simulink library "WECSim_Lib_Body_Elements"  (R2020b)
settings: Solver=VariableStepAuto  StartTime=0.0  StopTime=10.0  RelTol=1e-3
undefined symbols (not defined in the file or in its folder): body, simu, waves, X, Y, Z
libraries: nesl_utility x22, sm_lib x16, $bdroot x9, vrlib x3
(part 2 of 5)

== system WECSim_Lib_Body_Elements/Flex Body/Variable Hydrodynamics Control ==
  note: Developer note: When creating a new bus selector, it will only show the variables within hydroForce if they already exist in the workspace, which is inconventient. Copy this bus selector to more easily add calls to variables from hydroForce. This bus selector should already contains all variables in hydroForce which can then be selected, and extras deleted.
      |
      | Alternatively, open the bus selector block and use programmatic commands to set the output variables, e.g.
      | >> set_param(gcb, 'OutputSignals', 'storage.mass, volume');
  Bus Selector : BusSelector  Commented=on  OutputSignals=linearHydroRestCoef,storage,quadDrag,linearDamping,fExt,fExt.re,fExt.im,fExt.md,fAddedMass,fDamping,irkb,storage.mass,storage.inertia,storage.inertiaProducts,storage.fAddedMass,userDefinedFe,totDOF,fExt.dofGrd,fExt.dirGrd,fExt.wGrd,fExt.fEHRE,fExt.fEHIM,fExt.fEHMD
  Constant : Constant  Value=body.hydroForce  VectorParams1D=off  OutDataTypeStr=Bus: bus_body1_hydroForce
  From : From  Commented=on  GotoTag=body1_hydroForce
  Variable Hydrodynamics Subsystem : Subsystem  Variant=on  VariantControl=sv_b1_variableHydro  mask{body=body}
  tag scope: body1_hydroForce=global
  wires:
  Constant/1 -> Variable Hydrodynamics Subsystem/1(all_hydroForce)
  Variable Hydrodynamics Subsystem/1(selected_hydroForce) -> [body1_hydroForce]
  From/1 -> Bus Selector/1

== system WECSim_Lib_Body_Elements/Flex Body/Wave Diffraction and Excitation Force Calculation ==
  note: Do not link the `Wave Diffraction and Excitation Force Calculation`
      | to the rigid body block, this will break the Flex Body block.
  Time : Inport
  Displacement : Inport  Port=2
  WaveElv : Inport  Port=3
  Selector : Selector  InputPortWidth=body.dof  IndexOptions=Index vector (dialog)  Indices=[1:6]  OutputSizes=1
  Selector1 : Selector  InputPortWidth=body.dof  IndexOptions=Index vector (dialog)  Indices=[7:body.dofEnd]  OutputSizes=1
  Wave Diffraction and Excitation Force Calculation : Subsystem  mask{waveGroup=0}
      mask prompts: waveGroup "Waves Object"
      mask init:
      | cb = gcb;
      | nWaves = size(waveGroup,2);
      | for iWG = 2:nWaves
      |     try 
      |         find_system([cb,'/Linear Wave Excitation Force Variant Subsystem',num2str(iWG)],'Type','Block');
      |     catch
      |         add_block([cb,'/Linear Wave Excitation Force Variant Subsystem'],[cb,'/Wave Diffraction and Excitation Force Calculation/Linear Wave Excitation Force Variant Subsystem',num2str(iWG)],'MakeNameUnique','off',...
      |                    'Position',[400,200*iWG,580,40+200*iWG],'BackgroundColor','white');
      |         set_param([cb,'/Linear Wave Excitation Force Variant Subsystem',num2str(iWG)],...
      |                'Nwave',sprintf('waves(%d)',iWG) );
      | 
      |         add_line(cb,...
      |            ['FexcInputs/1'],...
      |             ['Linear Wave Excitation Force Variant Subsystem',num2str(iWG),'/1'],...
      |             'autorouting','on');
      |            add_line(cb,...
      |            ['FexcInputs/2'],...
      |             ['Linear Wave Excitation Force Variant Subsystem',num2str(iWG),'/2'],...
      |             'autorouting','on');
      |         signlist = get_param([cb,'/Add'],'Inputs');   
      |         set_param([cb,'/Add'],'Inputs',[signlist,'+']);
      |         add_line(cb,...
      |         ['Linear Wave Excitation Force Variant Subsystem',num2str(iWG),'/1'],...
      |         sprintf('Add/%d',length(signlist)+1),...
      |         'autorouting','on');
      |     end
      | end
  F_Excitation_Rigid : Outport  PortDimensions=6
  F_Excitation_Flex : Outport  Port=2  PortDimensions=body.gbmDOF
  wires:
  Displacement/1 -> Wave Diffraction and Excitation Force Calculation/2(Displacement)
  WaveElv/1 -> Wave Diffraction and Excitation Force Calculation/3(WaveElv)
  Time/1 -> Wave Diffraction and Excitation Force Calculation/1(Time)
  Selector1/1 -> F_Excitation_Flex/1
  Selector/1 -> F_Excitation_Rigid/1
  Wave Diffraction and Excitation Force Calculation/1(F_Excitation) -> Selector/1, Selector1/1

== system WECSim_Lib_Body_Elements/Flex Body/Wave Radiation Forces Calculation ==
  Velocity : Inport
  Acceleration : Inport  Port=2
  Selector : Selector  InputPortWidth=body.dof  IndexOptions=Index vector (dialog)  Indices=[1:6]  OutputSizes=1
  Selector1 : Selector  InputPortWidth=body.dof  IndexOptions=Index vector (dialog)  Indices=[7:body.dofEnd]  OutputSizes=1
  Selector2 : Selector  InputPortWidth=body.dof  IndexOptions=Index vector (dialog)  Indices=[1:6]  OutputSizes=1
  Selector3 : Selector  InputPortWidth=body.dof  IndexOptions=Index vector (dialog)  Indices=[7:body.dofEnd]  OutputSizes=1
  Wave Radiation Forces Calculation : Subsystem  AncestorBlock=WECSim_Lib_Body_Elements/Rigid Body/Hydrodynamic Body/Wave Radiation Forces Calculation  mask{body=body}
      mask prompts: body "Body class:"
  F_RadiationDamping_Rigid : Outport  PortDimensions=6
  F_RadiationDamping_Flex : Outport  Port=2  PortDimensions=body.gbmDOF
  F_AddedMass_Rigid : Outport  Port=3  PortDimensions=6
  F_AddedMass_Flex : Outport  Port=4  PortDimensions=body.gbmDOF
  wires:
  Velocity/1 -> Wave Radiation Forces Calculation/1(Velocity)
  Acceleration/1 -> Wave Radiation Forces Calculation/2(Acceleration)
  Wave Radiation Forces Calculation/1(F_RadiationDamping) -> Selector1/1, Selector/1  "F_RadiationDamping"
  Selector1/1 -> F_RadiationDamping_Flex/1
  Selector/1 -> F_RadiationDamping_Rigid/1
  Selector3/1 -> F_AddedMass_Flex/1
  Selector2/1 -> F_AddedMass_Rigid/1
  Wave Radiation Forces Calculation/2(F_AddedMass) -> Selector2/1, Selector3/1  "F_AddedMass"

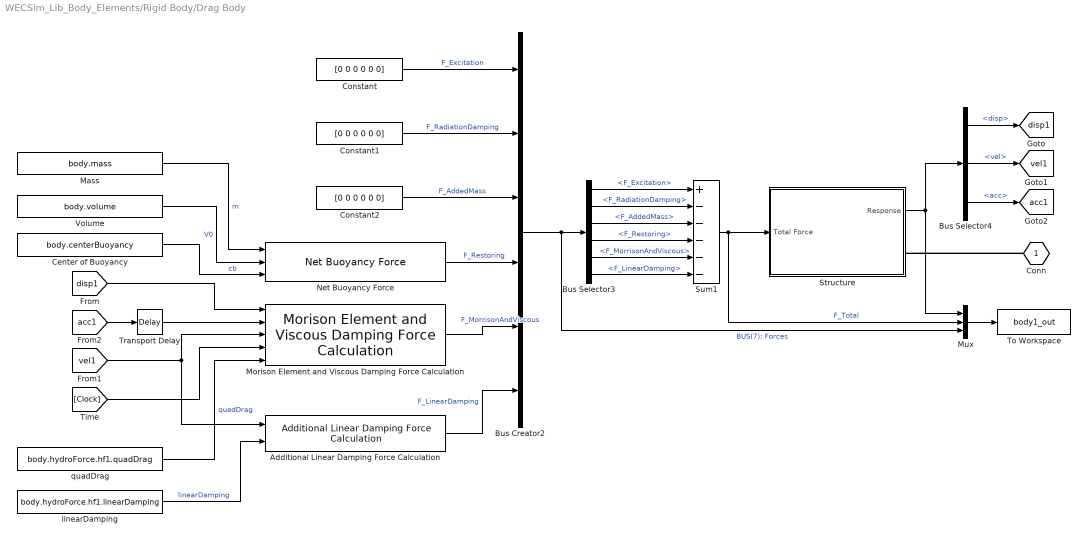
== system WECSim_Lib_Body_Elements/Rigid Body/Drag Body ==
  Additional Linear Damping Force Calculation : $bdroot/Rigid Body/Hydrodynamic Body/Additional Linear Damping Force Calculation  SystemSampleTime=-1  VariantActivationTime=update diagram  EmptyChoice=off  PassThrough=off  PassThroughVariantControl=(default)  EmptyChoiceVariantControl=(default)  Latency=0  AutoFrameSizeCalculation=off
  Bus Creator2 : BusCreator  Inputs=6
  Bus Selector3 : BusSelector  OutputSignals=F_Excitation,F_RadiationDamping,F_AddedMass,F_Restoring,F_MorrisonAndViscous,F_LinearDamping
  Bus Selector4 : BusSelector  OutputSignals=disp,vel,acc
  Center of Buoyancy : Constant  Value=body.centerBuoyancy
  Constant : Constant  Value=[0 0 0 0 0 0]
  Constant1 : Constant  Value=[0 0 0 0 0 0]
  Constant2 : Constant  Value=[0 0 0 0 0 0]
  Mass : Constant  Value=body.mass
  Morison Element and Viscous Damping Force Calculation : $bdroot/Rigid Body/Hydrodynamic Body/Morison Element and Viscous Damping Force Calculation  SystemSampleTime=-1  VariantActivationTime=update diagram  EmptyChoice=off  PassThrough=off  PassThroughVariantControl=(default)  EmptyChoiceVariantControl=(default)  Latency=0  AutoFrameSizeCalculation=off
  Mux : Mux  Inputs=3
  Net Buoyancy Force : $bdroot/Rigid Body/Hydrodynamic Body/Hydrostatic Restoring Force Calculation/Linear and Nonlinear Restoring Force Variant Subsystem/Linear Hydrostatic Restoring Force/Net Buoyancy Force  SystemSampleTime=-1  VariantActivationTime=update diagram  EmptyChoice=off  PassThrough=off  PassThroughVariantControl=(default)  EmptyChoiceVariantControl=(default)  Latency=0  AutoFrameSizeCalculation=off
  Structure : Subsystem
  Sum1 : Sum  Inputs=+-----
  To Workspace : ToWorkspace  VariableName=body1_out  SaveFormat=Structure With Time  SampleTime=simu.dtOut
  Transport Delay : TransportDelay  DelayTime=10e-8
  Volume : Constant  Value=body.volume
  linearDamping : Constant  Value=body.hydroForce.hf1.linearDamping
  quadDrag : Constant  Value=body.hydroForce.hf1.quadDrag
  Conn : PMIOPort  Side=Right
  tag scope: acc1=global, disp1=global, vel1=global
  wires:
  [acc1] -> Transport Delay/1
  Bus Selector3/1 -> Sum1/1  "<F_Excitation>"
  Bus Selector3/5 -> Sum1/5  "<F_MorrisonAndViscous>"
  Constant1/1 -> Bus Creator2/2  "F_RadiationDamping"
  Mux/1 -> To Workspace/1
  Net Buoyancy Force/1 -> Bus Creator2/4  "F_Restoring"
  Additional Linear Damping Force Calculation/1 -> Bus Creator2/6  "F_LinearDamping"
  Morison Element and Viscous Damping Force Calculation/1 -> Bus Creator2/5  "F_MorrisonAndViscous"
  Constant/1 -> Bus Creator2/1  "F_Excitation"
  Bus Selector3/4 -> Sum1/4  "<F_Restoring>"
  Bus Selector3/3 -> Sum1/3  "<F_AddedMass>"
  Bus Creator2/1 -> Mux/3, Bus Selector3/1  "BUS(7): Forces"
  Sum1/1 -> Mux/2, Structure/1(Total Force)  "F_Total"
  Constant2/1 -> Bus Creator2/3  "F_AddedMass"
  Bus Selector3/2 -> Sum1/2  "<F_RadiationDamping>"
  Bus Selector3/6 -> Sum1/6  "<F_LinearDamping>"
  Bus Selector4/1 -> [disp1]  "<disp>"
  Bus Selector4/2 -> [vel1]  "<vel>"
  Structure/1(Response) -> Mux/1, Bus Selector4/1
  Bus Selector4/3 -> [acc1]  "<acc>"
  Transport Delay/1 -> Morison Element and Viscous Damping Force Calculation/2
  [vel1] -> Morison Element and Viscous Damping Force Calculation/3, Additional Linear Damping Force Calculation/1
  [Clock] -> Morison Element and Viscous Damping Force Calculation/4
  [disp1] -> Morison Element and Viscous Damping Force Calculation/1
  Center of Buoyancy/1 -> Net Buoyancy Force/3  "cb"
  Volume/1 -> Net Buoyancy Force/2  "V0"
  Mass/1 -> Net Buoyancy Force/1  "m"
  quadDrag/1 -> Morison Element and Viscous Damping Force Calculation/5  "quadDrag"
  linearDamping/1 -> Additional Linear Damping Force Calculation/2  "linearDamping"
  connections:
  Conn/RConn1 -- Structure/RConn1

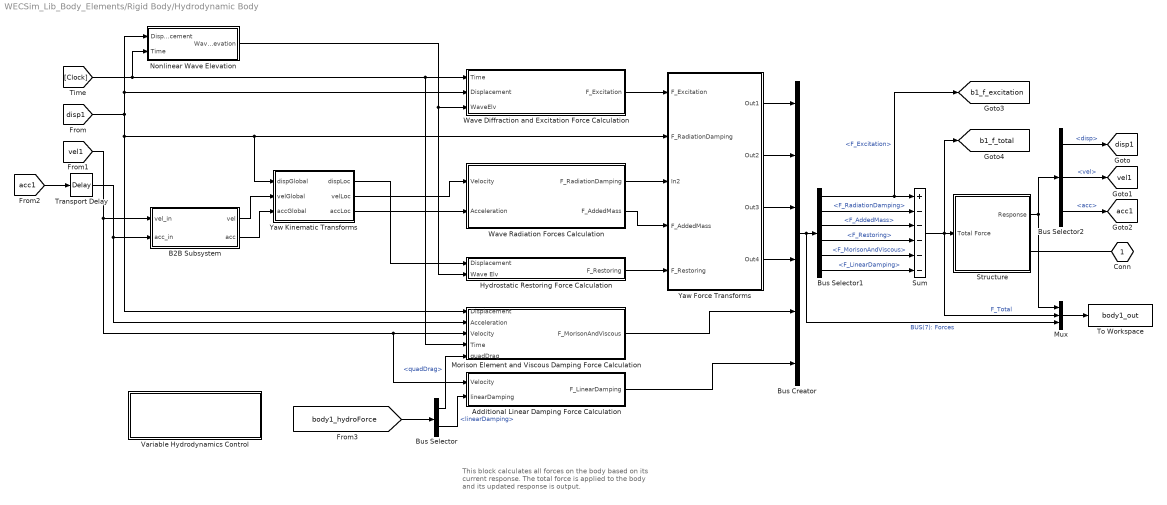
== system WECSim_Lib_Body_Elements/Rigid Body/Hydrodynamic Body ==
  note: This block calculates all forces on the body based on its current response. The total force is applied to the body and its updated response is output.
  Additional Linear Damping Force Calculation : Subsystem
  B2B Subsystem : Subsystem  Variant=on
  Bus Creator : BusCreator  Inputs=6
  Bus Selector : BusSelector  OutputSignals=quadDrag,linearDamping
  Bus Selector1 : BusSelector  OutputSignals=F_Excitation,F_RadiationDamping,F_AddedMass,F_Restoring,F_MorisonAndViscous,F_LinearDamping
  Bus Selector2 : BusSelector  OutputSignals=disp,vel,acc
  Hydrostatic Restoring Force Calculation : Subsystem
  Morison Element and Viscous Damping Force Calculation : Subsystem
  Mux : Mux  Inputs=3
  Nonlinear Wave Elevation : Subsystem  TreatAsAtomicUnit=on  SystemSampleTime=simu.nonlinearDt
  Structure : Subsystem
  Sum : Sum  Inputs=+-----
  To Workspace : ToWorkspace  VariableName=body1_out  SaveFormat=Structure With Time  SampleTime=simu.dtOut
  Transport Delay : TransportDelay  DelayTime=10e-8
  Variable Hydrodynamics Control : Subsystem  mask{body=body}
      mask prompts: body "Body Name:"
  Wave Diffraction and Excitation Force Calculation : Subsystem  mask{waveGroup=waves}
      mask prompts: waveGroup "Waves Object"
      mask init:
      | cb = gcb;
      | nWaves = size(waveGroup,2);
      | for iWG = 2:nWaves
      |     try 
      |         find_system([cb,'/Linear Wave Excitation Force Variant Subsystem',num2str(iWG)],'Type','Block');
      |     catch
      |         % Duplicate the linear excitation force block for multiple waves
      |         add_block([cb,'/Linear Wave Excitation Force Variant Subsystem'],[cb,'/Linear Wave Excitation Force Variant Subsystem',num2str(iWG)],'MakeNameUnique','off',...
      |                    'Position',[400,200*iWG,580,40+200*iWG],'BackgroundColor','white');
      |         set_param([cb,'/Linear Wave Excitation Force Variant Subsystem',num2str(iWG)],...
      |                'Nwave',sprintf('waves(%d)',iWG) );
      | 
      |         % Connect lines to the new block
      |         add_line(cb,...
      |            ['FexcInputs/1'],...
      |            ['Linear Wave Excitation Force Variant Subsystem',num2str(iWG),'/1'],...
      |            'autorouting','on');
      |         add_line(cb,...
      |            ['FexcInputs/2'],...
      |            ['Linear Wave Excitation Force Variant Subsystem',num2str(iWG),'/2'],...
      |            'autorouting','on');
      |         add_line(cb,...
      |            ['FexcInputs/4'],...
      |            ['Linear Wave Excitation Force Variant Subsystem',num2str(iWG),'/3'],...
      |            'autorouting','on');
      |         signlist = get_param([cb,'/Add'],'Inputs');   
      |         set_param([cb,'/Add'],'Inputs',[signlist,'+']);
      |         add_line(cb,...
      |         ['Linear Wave Excitation Force Variant Subsystem',num2str(iWG),'/1'],...
      |         sprintf('Add/%d',length(signlist)+1),...
      |         'autorouting','on');
      |     end
      | end
  Wave Radiation Forces Calculation : Subsystem
  Yaw Force Transforms : Subsystem
  Yaw Kinematic Transforms : Subsystem  Variant=on
  Conn : PMIOPort  Side=Right
  tag scope: acc1=global, b1_f_excitation=global, b1_f_total=global, disp1=global, vel1=global
  wires:
  Bus Selector1/6 -> Sum/6  "<F_LinearDamping>"
  Bus Selector1/5 -> Sum/5  "<F_MorisonAndViscous>"
  Bus Selector1/4 -> Sum/4  "<F_Restoring>"
  Bus Selector1/3 -> Sum/3  "<F_AddedMass>"
  Bus Selector1/2 -> Sum/2  "<F_RadiationDamping>"
  Bus Selector1/1 -> [b1_f_excitation], Sum/1  "<F_Excitation>"
  Hydrostatic Restoring Force Calculation/1(F_Restoring) -> Yaw Force Transforms/5(F_Restoring)
  [disp1] -> Nonlinear Wave Elevation/1(Displacement), Wave Diffraction and Excitation Force Calculation/2(Displacement), Yaw Kinematic Transforms/1(dispGlobal), Yaw Force Transforms/2(F_RadiationDamping), Morison Element and Viscous Damping Force Calculation/1(Displacement)
  Wave Diffraction and Excitation Force Calculation/1(F_Excitation) -> Yaw Force Transforms/1(F_Excitation)
  Wave Radiation Forces Calculation/2(F_AddedMass) -> Yaw Force Transforms/4(F_AddedMass)
  Morison Element and Viscous Damping Force Calculation/1(F_MorisonAndViscous) -> Bus Creator/5
  Structure/1(Response) -> Mux/1, Bus Selector2/1
  Bus Creator/1 -> Mux/3, Bus Selector1/1  "BUS(7): Forces"
  B2B Subsystem/2(acc) -> Yaw Kinematic Transforms/3(accGlobal)
  Bus Selector2/2 -> [vel1]  "<vel>"
  Sum/1 -> [b1_f_total], Mux/2, Structure/1(Total Force)  "F_Total"
  Bus Selector2/1 -> [disp1]  "<disp>"
  [acc1] -> Transport Delay/1
  Yaw Kinematic Transforms/3(accLoc) -> Wave Radiation Forces Calculation/2(Acceleration)
  [Clock] -> Nonlinear Wave Elevation/2(Time), Wave Diffraction and Excitation Force Calculation/1(Time), Morison Element and Viscous Damping Force Calculation/4(Time)
  Additional Linear Damping Force Calculation/1(F_LinearDamping) -> Bus Creator/6
  Transport Delay/1 -> B2B Subsystem/2(acc_in), Morison Element and Viscous Damping Force Calculation/2(Acceleration)
  Bus Selector2/3 -> [acc1]  "<acc>"
  B2B Subsystem/1(vel) -> Yaw Kinematic Transforms/2(velGlobal)
  Yaw Kinematic Transforms/1(dispLoc) -> Hydrostatic Restoring Force Calculation/1(Displacement)
  Yaw Kinematic Transforms/2(velLoc) -> Wave Radiation Forces Calculation/1(Velocity)
  Nonlinear Wave Elevation/1(Wave Elevation) -> Wave Diffraction and Excitation Force Calculation/3(WaveElv), Hydrostatic Restoring Force Calculation/2(Wave Elv)
  [vel1] -> B2B Subsystem/1(vel_in), Additional Linear Damping Force Calculation/1(Velocity), Morison Element and Viscous Damping Force Calculation/3(Velocity)
  Mux/1 -> To Workspace/1
  Wave Radiation Forces Calculation/1(F_RadiationDamping) -> Yaw Force Transforms/3(In2)
  Yaw Force Transforms/1(Out1) -> Bus Creator/1
  Yaw Force Transforms/2(Out2) -> Bus Creator/2
  Yaw Force Transforms/4(Out4) -> Bus Creator/4
  Yaw Force Transforms/3(Out3) -> Bus Creator/3
  [body1_hydroForce] -> Bus Selector/1
  Bus Selector/1 -> Morison Element and Viscous Damping Force Calculation/5(quadDrag)  "<quadDrag>"
  Bus Selector/2 -> Additional Linear Damping Force Calculation/2(linearDamping)  "<linearDamping>"
  connections:
  Conn/RConn1 -- Structure/RConn1

== system WECSim_Lib_Body_Elements/Flex Body/Hydrostatic Restoring Force Calculation/Hydrostatic Restoring Force Calculation ==
  Displacement : Inport
  Wave Elv : Inport  Port=2
  Add : Sum  Inputs=+-
  Bus Selector : BusSelector  OutputSignals=centerGravity
  Constant1 : Constant  Value=zeros(1,body.dof-3)
  Linear and Nonlinear Restoring Force Variant Subsystem : Subsystem  Variant=on
  Mux1 : Mux  Inputs=2
  F_Restoring : Outport
  wires:
  Displacement/1 -> Add/1  "x"
  Linear and Nonlinear Restoring Force Variant Subsystem/1(Out1) -> F_Restoring/1  "F_Restoring"
  Wave Elv/1 -> Linear and Nonlinear Restoring Force Variant Subsystem/2(In2)
  Add/1 -> Linear and Nonlinear Restoring Force Variant Subsystem/1(In1)  "x_cg"
  Constant1/1 -> Mux1/2
  Mux1/1 -> Add/2
  Bus Selector/1 -> Mux1/1  "<centerGravity>"
  [body1_hydroForce] -> Bus Selector/1

== system WECSim_Lib_Body_Elements/Flex Body/Variable Hydrodynamics Control/Variable Hydrodynamics Subsystem ==
  note: 1) Add Subsystem or Model blocks as valid variant choices.
      | 2) You cannot connect blocks at this level. At simulation, connectivity is automatically
      | determined, based on the active variant and port name matching.
  all_hydroForce : Inport
  noVariableHydro : Subsystem  VariantControl=sv_b1_noVariableHydro
  variableHydro : Subsystem  VariantControl=sv_b1_variableHydro  mask{body=body}
      mask prompts: body "Body Number:"
      mask init:
      | hydroForceElements = fields(body.hydroForce);
      | 
      | nElements = length(hydroForceElements);
      | elementString = hydroForceElements{1};
      | if nElements > 1
      |     for i=2:nElements
      |         elementString = [elementString ', ' hydroForceElements{i}]; 
      |     end
      | end
      | 
      | % delete previous lines
      | busSelectorBlock = Simulink.findBlocks(gcb,'BlockType','BusSelector');
      | lines = get_param(busSelectorBlock,'LineHandles');
      | for ii = 1:numel(lines.Outport)
      |     if lines.Outport(ii) ~= -1
      |         delete_line(lines.Outport(ii));
      |     end
      | end
      | 
      | % Update bus signals with the name of hydroForce elements (hf1, hf2, etc)
      | h = [gcb '/Bus Selector'];
      | set_param(h, 'OutputSignals', elementString);
      | 
      | % Update number of switch inputs
      | h = [gcb '/Multiport Switch'];
      | set_param(h, 'Inputs', num2str(nElements));
      | 
      | % Connect bus outputs and switch inputs
      | for i = 1:nElements
      |     try
      |         add_line(gcb, ...
      |             ['Bus Selector/' num2str(i)], ...
      |             ['Multiport Switch/' num2str(i+1)],...
      |             'autorouting','on');
      |     catch
      |     end
      | end
      | 
      | % Connect the initial case (default hydroForce) to the end of the multiport switch (default case)
      | hydroForceIndexInitial = body.variableHydro.hydroForceIndexInitial;
      | try
      |     add_line(gcb, ...
      |         ['Bus Selector/' num2str(hydroForceIndexInitial)], ...
      |         ['Multiport Switch/' num2str(nElements+2)],...
      |         'autorouting','on');
      | catch
      | end
  selected_hydroForce : Outport

== system WECSim_Lib_Body_Elements/Flex Body/Wave Diffraction and Excitation Force Calculation/Wave Diffraction and Excitation Force Calculation ==
  note: The excitation force = F_wave * ramp function
  Time : Inport
  Displacement : Inport  Port=2
  WaveElv : Inport  Port=3
  Add : Sum
  Constant : Constant
  FexcInputs : Subsystem
  Less Than : RelationalOperator  Operator=<  OutDataTypeStr=boolean  RndMeth=Simplest
  Linear Wave Excitation Force Variant Subsystem : Subsystem  Variant=on  mask{Nwave=waves(1)}
      mask prompts: Nwave "Wave Instance"
  Nonlinear FK Force Variant Subsystem : Subsystem  Variant=on
  Product : Product
  Ramp Function Time : Constant  Value=simu.rampTime
  Ramp function : Subsystem
  Switch : Switch  Criteria=u2 ~= 0
  F_Excitation : Outport  PortDimensions=body.dof
  wires:
  Ramp Function Time/1 -> Less Than/2
  Constant/1 -> Switch/3
  FexcInputs/1(Out1) -> Ramp function/1(Time), Less Than/1, Linear Wave Excitation Force Variant Subsystem/1(Time), Nonlinear FK Force Variant Subsystem/1(Time)
  Ramp function/1(R) -> Switch/1
  Less Than/1 -> Switch/2
  Nonlinear FK Force Variant Subsystem/1(Nonlinear Excitation) -> Add/2
  Linear Wave Excitation Force Variant Subsystem/1(Linear Excitation) -> Add/1
  FexcInputs/3(Out3) -> Nonlinear FK Force Variant Subsystem/3(WaveElv)
  FexcInputs/2(Out2) -> Nonlinear FK Force Variant Subsystem/2(Displacement), Linear Wave Excitation Force Variant Subsystem/2(Displacement)
  Product/1 -> F_Excitation/1  "F_Excitation"
  Add/1 -> Product/2  "F_wave"
  Switch/1 -> Product/1  "R"
  WaveElv/1 -> FexcInputs/3(WaveElv)
  Displacement/1 -> FexcInputs/2(Displacement)
  [body1_hydroForce] -> FexcInputs/4(body_hydroForce)
  Time/1 -> FexcInputs/1(Time)
  FexcInputs/4(Out4) -> Linear Wave Excitation Force Variant Subsystem/3(body_hydroForce)

== system WECSim_Lib_Body_Elements/Flex Body/Wave Radiation Forces Calculation/Wave Radiation Forces Calculation ==
  note: F_AddedMass = AM * a
  Velocity : Inport
  Acceleration : Inport  Port=2
  Bus Selector : BusSelector  OutputSignals=fAddedMass
  Product1 : Product  Multiplication=Matrix(*)
  SS CI and Constant-Damping-CoeVariant Subsystem : Subsystem  Variant=on
  F_RadiationDamping : Outport
  F_AddedMass : Outport  Port=2
  wires:
  Bus Selector/1 -> Product1/1  "<fAddedMass>"
  [body1_hydroForce] -> Bus Selector/1
  Acceleration/1 -> Product1/2
  SS CI and Constant-Damping-CoeVariant Subsystem/1(Out1) -> F_RadiationDamping/1  "F_RadiationDamping"
  Velocity/1 -> SS CI and Constant-Damping-CoeVariant Subsystem/1(velocity)
  Product1/1 -> F_AddedMass/1  "F_AddedMass"

== system WECSim_Lib_Body_Elements/Rigid Body/Drag Body/Structure ==
  note: Apply the total force to the body and calculate its response relative to the global reference frame.
      |
      | Output force to apply to another body.
  Total Force : Inport
  Body Properties : sm_lib/Body Elements/File Solid  ExtGeomFileName=geometry/float.stl  UnitType=Custom  ExtGeomFileUnits=m  StepReaderType=HEX  ExportConvexHullGeometry=off  InertiaType=Custom  BasedOnType=Density  Density=1000  DensityUnits=kg/(m^3)  Mass=body.mass  MassUnits=kg  CenterOfMass=[0 0 0]  CenterOfMassUnits=m  MomentsOfInertia=body.inertia  MomentsOfInertiaUnits=kg*m^2  ProductsOfInertia=body.inertiaProducts  ProductsOfInertiaUnits=kg*m^2  GraphicType=FromGeometry  MarkerShape=Sphere  MarkerSize=10  GraphicVisPropType=SimpleVisualProperties  GraphicDiffuseColor=body.viz.color  GraphicOpacity=body.viz.opacity  GraphicSpecularColor=[0.5 0.5 0.5 1.0]  GraphicAmbientColor=[0.15 0.15 0.15 1.0]  GraphicEmissiveColor=[0.0 0.0 0.0 1.0]  GraphicShininess=75  DoExposeReferenceFrame=on  SerializedFrames=<Frames/>
  External Force and Torque : sm_lib/Forces and Torques/External Force and Torque  EnableForceX=off  EnableForceY=off  EnableForceZ=off  EnableForce=on  ForceResolutionFrame=World  EnableTorqueX=off  EnableTorqueY=off  EnableTorqueZ=off  EnableTorque=on  TorqueResolutionFrame=World
  Motion Sensor : $bdroot/Rigid Body/Hydrodynamic Body/Structure/Motion Sensor  SystemSampleTime=-1  VariantActivationTime=update diagram  EmptyChoice=off  PassThrough=off  PassThroughVariantControl=(default)  EmptyChoiceVariantControl=(default)  Latency=0  AutoFrameSizeCalculation=off
  Rigid Transform (Setup CG) : sm_lib/Frames and Transforms/Rigid Transform  RotationMethod=None  FollAlignAxisA=+X  BaseAlignAxisA=+Y  FollAlignAxisB=+Y  BaseAlignAxisB=+Z  RotationStandardAxis=+Y  RotationAngle=0.05  RotationAngleUnits=rad  RotationArbitraryAxis=[0.57735026918962584 0.57735026918962584 0.57735026918962584]  RotationSequenceAxes=FollowerAxes  RotationSequence=XYX  RotationSequenceAngles=[0 0 0]  RotationSequenceAnglesUnits=deg  RotationMatrix=[1 0 0; 0 1 0; 0 0 1]  Quaternion=[1 0 0 0]  TranslationMethod=Cartesian  TranslationCartesianOffset=body.centerGravity  TranslationCartesianOffsetUnits=m  TranslationStandardAxis=+Z  TranslationStandardOffset=0  TranslationStandardOffsetUnits=m  TranslationROffset=0  TranslationROffsetUnits=m  TranslationThetaOffset=0  TranslationThetaOffsetUnits=deg  TranslationZOffset=0  TranslationZOffsetUnits=m
  Rigid Transform (Setup Initial Disp) : sm_lib/Frames and Transforms/Rigid Transform  RotationMethod=ArbitraryAxis  FollAlignAxisA=+X  BaseAlignAxisA=+Y  FollAlignAxisB=+Y  BaseAlignAxisB=+Z  RotationStandardAxis=+Y  RotationAngle=body.initial.angle  RotationAngleUnits=rad  RotationArbitraryAxis=body.initial.axis  RotationSequenceAxes=FollowerAxes  RotationSequence=XYX  RotationSequenceAngles=[0 0 0]  RotationSequenceAnglesUnits=deg  RotationMatrix=[1 0 0; 0 1 0; 0 0 1]  Quaternion=[1 0 0 0]  TranslationMethod=Cartesian  TranslationCartesianOffset=body.initial.displacement  TranslationCartesianOffsetUnits=m  TranslationStandardAxis=+Z  TranslationStandardOffset=0  TranslationStandardOffsetUnits=m  TranslationROffset=0  TranslationROffsetUnits=m  TranslationThetaOffset=0  TranslationThetaOffsetUnits=deg  TranslationZOffset=0  TranslationZOffsetUnits=m
  Selector : Selector  InputPortWidth=6  IndexOptions=Index vector (dialog)  Indices=[1:3]  OutputSizes=1
  Selector1 : Selector  InputPortWidth=6  IndexOptions=Index vector (dialog)  Indices=[4:6]  OutputSizes=1
  Simulink-PS Converter1 : nesl_utility/Simulink-PS Converter  PhysicalDomain=network_engine_domain  SubClassName=ps_input  LeftPortType=input  RightPortType=output  PseudoPeriodic=off  Frequencies=[]  NoiseDistribution=none  NoiseParameters=[]  Unit=1  AffineConversion=off  FilteringAndDerivatives=zero  SimscapeFilterOrder=1  InputFilterTimeConstant=0.001  UdotUserProvided=1
  Simulink-PS Converter2 : nesl_utility/Simulink-PS Converter  PhysicalDomain=network_engine_domain  SubClassName=ps_input  LeftPortType=input  RightPortType=output  PseudoPeriodic=off  Frequencies=[]  NoiseDistribution=none  NoiseParameters=[]  Unit=1  AffineConversion=off  FilteringAndDerivatives=zero  SimscapeFilterOrder=1  InputFilterTimeConstant=0.001  UdotUserProvided=1
  World Frame : sm_lib/Frames and Transforms/World Frame
  Conn Free Surface : PMIOPort  Side=Right
  Response : Outport
  wires:
  Motion Sensor/1 -> Response/1
  Selector1/1 -> Simulink-PS Converter2/1
  Selector/1 -> Simulink-PS Converter1/1
  Total Force/1 -> Selector/1, Selector1/1
  connections:
  Motion Sensor/LConn1 -- World Frame/RConn1
  Rigid Transform (Setup Initial Disp)/LConn1 -- Rigid Transform (Setup CG)/RConn1
  Conn Free Surface/RConn1 -- Rigid Transform (Setup CG)/LConn1
  External Force and Torque/RConn1 -- Motion Sensor/RConn1 -- Body Properties/RConn1 -- Rigid Transform (Setup Initial Disp)/RConn1
  External Force and Torque/LConn2 -- Simulink-PS Converter2/RConn1
  External Force and Torque/LConn1 -- Simulink-PS Converter1/RConn1

== system WECSim_Lib_Body_Elements/Rigid Body/Hydrodynamic Body/Additional Linear Damping Force Calculation ==
  note: F_damping = c*v
  Velocity : Inport
  linearDamping : Inport  Port=2
  Product1 : Product  Multiplication=Matrix(*)
  F_LinearDamping : Outport
  wires:
  Product1/1 -> F_LinearDamping/1  "F_LinearDamping"
  Velocity/1 -> Product1/2  "v"
  linearDamping/1 -> Product1/1

== system WECSim_Lib_Body_Elements/Rigid Body/Hydrodynamic Body/B2B Subsystem ==
  note: If simu.b2b == 0, no body to body interaction is used (noB2B)
      | If simu.b2b == 1, use body to body interaction (B2B)
  note: 1) Add Subsystem or Model blocks as valid variant choices.
      | 2) You cannot connect blocks at this level. At simulation, connectivity is automatically
      | determined, based on the active variant and port name matching.
  vel_in : Inport
  acc_in : Inport  Port=2
  B2B : Subsystem  VariantControl=sv_B2B
  noB2B : Subsystem  VariantControl=sv_noB2B
  vel : Outport
  acc : Outport  Port=2

== system WECSim_Lib_Body_Elements/Rigid Body/Hydrodynamic Body/Hydrostatic Restoring Force Calculation ==
  Displacement : Inport
  Wave Elv : Inport  Port=2
  Add : Sum  Inputs=+-
  Bus Selector : BusSelector  OutputSignals=centerGravity
  Constant : Constant  Value=zeros(1,body.dof-3)
  Linear and Nonlinear Restoring Force Variant Subsystem : Subsystem  Variant=on
  Mux : Mux  Inputs=2
  F_Restoring : Outport
  wires:
  Displacement/1 -> Add/1  "x"
  Linear and Nonlinear Restoring Force Variant Subsystem/1(Out1) -> F_Restoring/1  "F_Restoring"
  Mux/1 -> Add/2
  Bus Selector/1 -> Mux/1  "<centerGravity>"
  Constant/1 -> Mux/2
  Wave Elv/1 -> Linear and Nonlinear Restoring Force Variant Subsystem/2(In2)
  Add/1 -> Linear and Nonlinear Restoring Force Variant Subsystem/1(In1)  "x_cg"
  [body1_hydroForce] -> Bus Selector/1

== system WECSim_Lib_Body_Elements/Rigid Body/Hydrodynamic Body/Morison Element and Viscous Damping Force Calculation ==
  note: The output force is a combination of the quadratic viscous drag force and the Morison element force.
      |
      | F_quadraticViscous = 0.5*Cd*rho*A*v*|v|
  Displacement : Inport
  Acceleration : Inport  Port=2
  Velocity : Inport  Port=3
  Time : Inport  Port=4
  quadDrag : Inport  Port=5
  Abs1 : Abs
  Morison Element Variant Subsystem : Subsystem  Variant=on
  Product : Product
  Product1 : Product  Multiplication=Matrix(*)
  Transport Delay : TransportDelay  DelayTime=10e-8
  "VisSum " : Sum  Inputs=+-
  F_MorisonAndViscous : Outport
  wires:
  "VisSum "/1 -> F_MorisonAndViscous/1  "F_MorisonAndViscous"
  Acceleration/1 -> Transport Delay/1
  Abs1/1 -> Product/2
  Product1/1 -> "VisSum "/1  "F_quadraticViscous"
  Product/1 -> Product1/2  "v * |v|"
  Time/1 -> Morison Element Variant Subsystem/4(time)
  Displacement/1 -> Morison Element Variant Subsystem/1(displacement)
  Transport Delay/1 -> Morison Element Variant Subsystem/3(acceleration)
  Velocity/1 -> Product/1, Morison Element Variant Subsystem/2(velocity), Abs1/1
  Morison Element Variant Subsystem/1(morison_force) -> "VisSum "/2
  quadDrag/1 -> Product1/1  "quadDrag = 0.5 * cd * rho *A"

== system WECSim_Lib_Body_Elements/Rigid Body/Hydrodynamic Body/Nonlinear Wave Elevation ==
  Displacement : Inport
  Time : Inport  Port=2
  Add : Sum  Inputs=+-
  Center of Gravity : Constant  Value=body.centerGravity
  Constant : Constant  Value=zeros(1,body.dof-3)
  Linear or Instantaneous Free Surface : Subsystem  Variant=on
  Mux : Mux  Inputs=2
  Wave Elevation : Outport
  wires:
  Displacement/1 -> Add/1  "x"
  Linear or Instantaneous Free Surface/1(Out1) -> Wave Elevation/1
  Add/1 -> Linear or Instantaneous Free Surface/1(In1)  "x_cg"
  Mux/1 -> Add/2
  Center of Gravity/1 -> Mux/1  "cg"
  Constant/1 -> Mux/2
  Time/1 -> Linear or Instantaneous Free Surface/2(In2)

== system WECSim_Lib_Body_Elements/Rigid Body/Hydrodynamic Body/Structure ==
  note: Apply the total force to the body and calculate its response relative to the global reference frame.
      |
      | Output force to apply to another body.
  Total Force : Inport
  Body Properties : sm_lib/Body Elements/File Solid  ExtGeomFileName=geometry/float.stl  UnitType=Custom  ExtGeomFileUnits=m  StepReaderType=HEX  ExportConvexHullGeometry=off  InertiaType=Custom  BasedOnType=Density  Density=1000  DensityUnits=kg/(m^3)  Mass=body.hydroForce.(['hf' num2str(body.variableHydro.hydroForceIndexInitial)]).adjustedMass  MassUnits=kg  CenterOfMass=[0 0 0]  CenterOfMassUnits=m  MomentsOfInertia=body.hydroForce.(['hf' num2str(body.variableHydro.hydroForceIndexInitial)]).adjustedInertia  MomentsOfInertiaUnits=kg*m^2  ProductsOfInertia=body.hydroForce.(['hf' num2str(body.variableHydro.hydroForceIndexInitial)]).adjustedInertiaProducts  ProductsOfInertiaUnits=kg*m^2  GraphicType=FromGeometry  MarkerShape=Sphere  MarkerSize=10  GraphicVisPropType=SimpleVisualProperties  GraphicDiffuseColor=body.viz.color  GraphicOpacity=body.viz.opacity  GraphicSpecularColor=[0.5 0.5 0.5 1.0]  GraphicAmbientColor=[0.15 0.15 0.15 1.0]  GraphicEmissiveColor=[0.0 0.0 0.0 1.0]  GraphicShininess=75  DoExposeReferenceFrame=on  SerializedFrames=<Frames/>
  External Force and Torque : sm_lib/Forces and Torques/External Force and Torque  EnableForceX=off  EnableForceY=off  EnableForceZ=off  EnableForce=on  ForceResolutionFrame=World  EnableTorqueX=off  EnableTorqueY=off  EnableTorqueZ=off  EnableTorque=on  TorqueResolutionFrame=World
  Motion Sensor : Subsystem
  Rigid Transform (Setup CG) : sm_lib/Frames and Transforms/Rigid Transform  RotationMethod=None  FollAlignAxisA=+X  BaseAlignAxisA=+Y  FollAlignAxisB=+Y  BaseAlignAxisB=+Z  RotationStandardAxis=+Y  RotationAngle=0.05  RotationAngleUnits=rad  RotationArbitraryAxis=[0.57735026918962584 0.57735026918962584 0.57735026918962584]  RotationSequenceAxes=FollowerAxes  RotationSequence=XYX  RotationSequenceAngles=[0 0 0]  RotationSequenceAnglesUnits=deg  RotationMatrix=[1 0 0; 0 1 0; 0 0 1]  Quaternion=[1 0 0 0]  TranslationMethod=Cartesian  TranslationCartesianOffset=body.centerGravity  TranslationCartesianOffsetUnits=m  TranslationStandardAxis=+Z  TranslationStandardOffset=0  TranslationStandardOffsetUnits=m  TranslationROffset=0  TranslationROffsetUnits=m  TranslationThetaOffset=0  TranslationThetaOffsetUnits=deg  TranslationZOffset=0  TranslationZOffsetUnits=m
  Rigid Transform (Setup Initial Disp) : sm_lib/Frames and Transforms/Rigid Transform  RotationMethod=ArbitraryAxis  FollAlignAxisA=+X  BaseAlignAxisA=+Y  FollAlignAxisB=+Y  BaseAlignAxisB=+Z  RotationStandardAxis=+Y  RotationAngle=body.initial.angle  RotationAngleUnits=rad  RotationArbitraryAxis=body.initial.axis  RotationSequenceAxes=FollowerAxes  RotationSequence=XYX  RotationSequenceAngles=[0 0 0]  RotationSequenceAnglesUnits=deg  RotationMatrix=[1 0 0; 0 1 0; 0 0 1]  Quaternion=[1 0 0 0]  TranslationMethod=Cartesian  TranslationCartesianOffset=body.initial.displacement  TranslationCartesianOffsetUnits=m  TranslationStandardAxis=+Z  TranslationStandardOffset=0  TranslationStandardOffsetUnits=m  TranslationROffset=0  TranslationROffsetUnits=m  TranslationThetaOffset=0  TranslationThetaOffsetUnits=deg  TranslationZOffset=0  TranslationZOffsetUnits=m
  Selector : Selector  InputPortWidth=6  IndexOptions=Index vector (dialog)  Indices=[1:3]  OutputSizes=1
  Selector1 : Selector  InputPortWidth=6  IndexOptions=Index vector (dialog)  Indices=[4:6]  OutputSizes=1
  Simulink-PS Converter1 : nesl_utility/Simulink-PS Converter  PhysicalDomain=network_engine_domain  SubClassName=ps_input  LeftPortType=input  RightPortType=output  PseudoPeriodic=off  Frequencies=[]  NoiseDistribution=none  NoiseParameters=[]  Unit=1  AffineConversion=off  FilteringAndDerivatives=zero  SimscapeFilterOrder=1  InputFilterTimeConstant=0.001  UdotUserProvided=1
  Simulink-PS Converter2 : nesl_utility/Simulink-PS Converter  PhysicalDomain=network_engine_domain  SubClassName=ps_input  LeftPortType=input  RightPortType=output  PseudoPeriodic=off  Frequencies=[]  NoiseDistribution=none  NoiseParameters=[]  Unit=1  AffineConversion=off  FilteringAndDerivatives=zero  SimscapeFilterOrder=1  InputFilterTimeConstant=0.001  UdotUserProvided=1
  World Frame : sm_lib/Frames and Transforms/World Frame
  Conn Free Surface : PMIOPort  Side=Right
  Response : Outport
  wires:
  Motion Sensor/1(Response) -> Response/1
  Selector1/1 -> Simulink-PS Converter2/1
  Selector/1 -> Simulink-PS Converter1/1
  Total Force/1 -> Selector/1, Selector1/1
  connections:
  World Frame/RConn1 -- Motion Sensor/LConn1
  Rigid Transform (Setup Initial Disp)/LConn1 -- Rigid Transform (Setup CG)/RConn1
  Conn Free Surface/RConn1 -- Rigid Transform (Setup CG)/LConn1
  Motion Sensor/RConn1 -- External Force and Torque/RConn1 -- Body Properties/RConn1 -- Rigid Transform (Setup Initial Disp)/RConn1
  External Force and Torque/LConn2 -- Simulink-PS Converter2/RConn1
  External Force and Torque/LConn1 -- Simulink-PS Converter1/RConn1

== system WECSim_Lib_Body_Elements/Rigid Body/Hydrodynamic Body/Variable Hydrodynamics Control ==
  note: Developer note: When creating a new bus selector, it will only show the variables within hydroForce if they already exist in the workspace, which is inconventient. Copy this bus selector to more easily add calls to variables from hydroForce. This bus selector should already contains all variables in hydroForce which can then be selected, and extras deleted.
      |
      | Alternatively, open the bus selector block and use programmatic commands to set the output variables, e.g.
      | >> set_param(gcb, 'OutputSignals', 'storage.mass, volume');
  Bus Selector : BusSelector  Commented=on  OutputSignals=linearHydroRestCoef,storage,quadDrag,linearDamping,fExt,fExt.re,fExt.im,fExt.md,fAddedMass,fDamping,irkb,storage.mass,storage.inertia,storage.inertiaProducts,storage.fAddedMass,userDefinedFe,totDOF,fExt.dofGrd,fExt.dirGrd,fExt.wGrd,fExt.fEHRE,fExt.fEHIM,fExt.fEHMD
  Constant : Constant  Value=body.hydroForce  VectorParams1D=off  OutDataTypeStr=Bus: bus_body1_hydroForce
  From : From  Commented=on  GotoTag=body1_hydroForce
  Variable Hydrodynamics Subsystem : Subsystem  Variant=on  VariantControl=sv_b1_variableHydro  mask{body=body}
  tag scope: body1_hydroForce=global
  wires:
  Constant/1 -> Variable Hydrodynamics Subsystem/1(all_hydroForce)
  Variable Hydrodynamics Subsystem/1(selected_hydroForce) -> [body1_hydroForce]
  From/1 -> Bus Selector/1

== system WECSim_Lib_Body_Elements/Rigid Body/Hydrodynamic Body/Wave Diffraction and Excitation Force Calculation ==
  note: The excitation force = F_wave * ramp function
  Time : Inport
  Displacement : Inport  Port=2
  WaveElv : Inport  Port=3
  Add : Sum  Inputs=+++
  Constant : Constant
  FexcInputs : Subsystem
  Less Than : RelationalOperator  Operator=<  OutDataTypeStr=boolean  RndMeth=Simplest
  Linear Wave Excitation Force Variant Subsystem : Subsystem  Variant=on  VariantControl=sv_irregularWavesNonLinYaw_b1  mask{Nwave=waves(1)}
      mask prompts: Nwave "Wave Instance"
  Nonlinear FK Force Variant Subsystem : Subsystem  Variant=on
  Product : Product
  Ramp Function Time : Constant  Value=simu.rampTime
  Ramp function : Subsystem
  Second Order Excitation Force Variant Subsystem : Subsystem  Variant=on
  Switch : Switch  Criteria=u2 ~= 0
  F_Excitation : Outport  PortDimensions=body.dof
  wires:
  Switch/1 -> Product/1  "R"
  Add/1 -> Product/2  "F_wave"
  Product/1 -> F_Excitation/1  "F_Excitation"
  Linear Wave Excitation Force Variant Subsystem/1(Linear Excitation) -> Add/1
  Nonlinear FK Force Variant Subsystem/1(Nonlinear Excitation) -> Add/2
  Ramp Function Time/1 -> Less Than/2
  Ramp function/1(R) -> Switch/1
  Less Than/1 -> Switch/2
  Constant/1 -> Switch/3
  FexcInputs/2(Out2) -> Linear Wave Excitation Force Variant Subsystem/2(Displacement), Second Order Excitation Force Variant Subsystem/3(displacement), Nonlinear FK Force Variant Subsystem/2(Displacement)
  Time/1 -> FexcInputs/1(Time)
  Displacement/1 -> FexcInputs/2(Displacement)
  WaveElv/1 -> FexcInputs/3(WaveElv)
  FexcInputs/3(Out3) -> Nonlinear FK Force Variant Subsystem/3(WaveElv)
  FexcInputs/1(Out1) -> Second Order Excitation Force Variant Subsystem/1(Time), Linear Wave Excitation Force Variant Subsystem/1(Time), Ramp function/1(Time), Less Than/1, Nonlinear FK Force Variant Subsystem/1(Time)
  Second Order Excitation Force Variant Subsystem/1(Second Order Excitation) -> Add/3
  FexcInputs/4(Out4) -> Linear Wave Excitation Force Variant Subsystem/3(body_hydroForce), Second Order Excitation Force Variant Subsystem/2(body_hydroForce)
  [body1_hydroForce] -> FexcInputs/4(body_hydroForce)

== system WECSim_Lib_Body_Elements/Rigid Body/Hydrodynamic Body/Wave Radiation Forces Calculation ==
  note: F_AddedMass = AM * a
  Velocity : Inport
  Acceleration : Inport  Port=2
  Bus Selector : BusSelector  OutputSignals=fAddedMass
  Product1 : Product  Multiplication=Matrix(*)
  SS CI and Constant-Damping-CoeVariant Subsystem : Subsystem  Variant=on
  F_RadiationDamping : Outport
  F_AddedMass : Outport  Port=2
  wires:
  Product1/1 -> F_AddedMass/1  "F_AddedMass"
  Velocity/1 -> SS CI and Constant-Damping-CoeVariant Subsystem/1(velocity)
  SS CI and Constant-Damping-CoeVariant Subsystem/1(Out1) -> F_RadiationDamping/1  "F_RadiationDamping"
  Acceleration/1 -> Product1/2
  [body1_hydroForce] -> Bus Selector/1
  Bus Selector/1 -> Product1/1  "<fAddedMass>"

== system WECSim_Lib_Body_Elements/Rigid Body/Hydrodynamic Body/Yaw Force Transforms ==
  F_Excitation : Inport
  F_RadiationDamping : Inport  Port=2
  In2 : Inport  Port=3
  F_AddedMass : Inport  Port=4
  F_Restoring : Inport  Port=5
  Constant : Constant  Value=body.yaw.option
  Yaw Force Transforms : MATLAB Function  TreatAsAtomicUnit=on
  Out1 : Outport
  Out2 : Outport  Port=2
  Out3 : Outport  Port=3
  Out4 : Outport  Port=4
  wires:
  Constant/1 -> Yaw Force Transforms/1(yaw)
  F_Restoring/1 -> Yaw Force Transforms/6(F_RestoringLocal)
  In2/1 -> Yaw Force Transforms/3(F_RadiationDampingLocal)
  F_Excitation/1 -> Yaw Force Transforms/5(F_ExcitationLocal)
  Yaw Force Transforms/4(F_Restoring) -> Out4/1
  F_AddedMass/1 -> Yaw Force Transforms/4(F_AddedMassLocal)
  F_RadiationDamping/1 -> Yaw Force Transforms/2(dispGlobal)
  Yaw Force Transforms/2(F_RadiationDamping) -> Out2/1
  Yaw Force Transforms/3(F_AddedMass) -> Out3/1
  Yaw Force Transforms/1(F_Excitation) -> Out1/1

== system WECSim_Lib_Body_Elements/Rigid Body/Hydrodynamic Body/Yaw Kinematic Transforms ==
  note: 1) Add Subsystem or Model blocks as valid variant choices.
      | 2) You cannot connect blocks at this level. At simulation, connectivity is automatically
      | determined, based on the active variant and port name matching.
  note: If simu.b2b == 0, no body to body interaction is used (noB2B)
      | If simu.b2b == 1, use body to body interaction (B2B)
  dispGlobal : Inport
  velGlobal : Inport  Port=2
  accGlobal : Inport  Port=3
  No B2B : Subsystem  VariantControl=sv_noB2B
  With B2B : Subsystem  VariantControl=sv_B2B
  dispLoc : Outport
  velLoc : Outport  Port=2
  accLoc : Outport  Port=3

== system WECSim_Lib_Body_Elements/Flex Body/Hydrostatic Restoring Force Calculation/Hydrostatic Restoring Force Calculation/Linear and Nonlinear Restoring Force Variant Subsystem ==
  note: If simu.nlHydro == 0, use the linear force option.
      | If simu.nlHydro > 0, use the nonlinear force option.
  note: 1) Add Subsystem or Model blocks as valid variant choices.
      | 2) You cannot connect blocks at this level. At simulation, connectivity is automatically
      | determined, based on the active variant and port name matching.
  In1 : Inport
  In2 : Inport  Port=2
  Linear Hydrostatic Restoring Force : Subsystem  VariantControl=sv_b1_linearHydro
  Nonlinear Hydrostatic Restoring Force : Subsystem  VariantControl=sv_b1_nonlinearHydro
  Out1 : Outport

== system WECSim_Lib_Body_Elements/Flex Body/Variable Hydrodynamics Control/Variable Hydrodynamics Subsystem/noVariableHydro ==
  all_hydroForce : Inport
  Bus Selector : BusSelector  OutputSignals=hf1
  selected_hydroForce : Outport
  wires:
  Bus Selector/1 -> selected_hydroForce/1  "<hf1>"
  all_hydroForce/1 -> Bus Selector/1  "x"

== system WECSim_Lib_Body_Elements/Flex Body/Variable Hydrodynamics Control/Variable Hydrodynamics Subsystem/variableHydro ==
  all_hydroForce : Inport
  Bus Selector : BusSelector  OutputSignals=hf1
  Multiport Switch : MultiPortSwitch  Inputs=1  DataPortForDefault=Additional data port  DiagnosticForDefault=Warning  OutDataTypeStr=Inherit: Same as first data input  RndMeth=Round
      settings: LockScale=on
  To Workspace : ToWorkspace  VariableName=body1_hydroForceIndex  SaveFormat=Structure With Time  SampleTime=simu.dtOut
  selected_hydroForce : Outport
  wires:
  all_hydroForce/1 -> Bus Selector/1
  [body1_hydroForceIndex] -> To Workspace/1, Multiport Switch/1
  Multiport Switch/1 -> selected_hydroForce/1
  Bus Selector/1 -> Multiport Switch/2  "<hf1>"

== system WECSim_Lib_Body_Elements/Flex Body/Wave Diffraction and Excitation Force Calculation/Wave Diffraction and Excitation Force Calculation/FexcInputs ==
  Time : Inport
  Displacement : Inport  Port=2
  WaveElv : Inport  Port=3
  body_hydroForce : Inport  Port=4
  Out1 : Outport
  Out2 : Outport  Port=2
  Out3 : Outport  Port=3
  Out4 : Outport  Port=4
  wires:
  WaveElv/1 -> Out3/1
  Time/1 -> Out1/1
  Displacement/1 -> Out2/1
  body_hydroForce/1 -> Out4/1

== system WECSim_Lib_Body_Elements/Flex Body/Wave Diffraction and Excitation Force Calculation/Wave Diffraction and Excitation Force Calculation/Linear Wave Excitation Force Variant Subsystem ==
  note: 1) Add Subsystem or Model blocks as valid variant choices.
      | 2) You cannot connect blocks at this level. At simulation, connectivity is automatically
      | determined, based on the active variant and port name matching.
  note: No wave includes wave.type == 'noWave' or 'noWaveCIC'
      | Regular wave includes wave.type == 'regular' or 'regularCIC'
      | Irregular wave includes wave.type == 'irregular' or 'spectrumImport'
  Time : Inport
  Displacement : Inport  Port=2
  body_hydroForce : Inport  Port=3
  Irregular Wave Excitation Force : Subsystem  VariantControl=sv_irregularWaves_b1
  Irregular Wave NonLinearYaw : Subsystem  VariantControl=sv_irregularWavesYaw_b1
  Irregular Wave Full Direction : Subsystem  VariantControl=sv_fullDirIrregularWaves_b1
  No Wave Excitation Force : Subsystem  VariantControl=sv_noWave
  Regular Wave Excitation Force : Subsystem  VariantControl=sv_regularWaves_b1
  Regular Wave NonLinear Yaw : Subsystem  VariantControl=sv_regularWavesYaw_b1
  User Defined Wave Excitation Force : Subsystem  VariantControl=sv_udfWaves
  Linear Excitation : Outport

== system WECSim_Lib_Body_Elements/Flex Body/Wave Diffraction and Excitation Force Calculation/Wave Diffraction and Excitation Force Calculation/Nonlinear FK Force Variant Subsystem ==
  note: 1) Add Subsystem or Model blocks as valid variant choices.
      | 2) You cannot connect blocks at this level. At simulation, connectivity is automatically
      | determined, based on the active variant and port name matching.
  note: If simu.nlHydro == 0, use No Nonlinear FroudeKrylov force option (nonlinear force is zero),
      | If simu.nlHydro > 0, use the Nonlinear FroudeKrylov force option,
  Time : Inport
  Displacement : Inport  Port=2
  WaveElv : Inport  Port=3
  No Nonlinear FroudeKrylov Force : Subsystem  VariantControl=sv_b1_linearHydro
  With Nonlinear FroudeKrylov Force : Subsystem  TreatAsAtomicUnit=on  SystemSampleTime=simu.nonlinearDt  VariantControl=sv_b1_nonlinearHydro
  Nonlinear Excitation : Outport

== system WECSim_Lib_Body_Elements/Flex Body/Wave Diffraction and Excitation Force Calculation/Wave Diffraction and Excitation Force Calculation/Ramp function ==
  note: The ramp function R, is a smooth function:
      | R = (sin(3*pi/2 + pi * t/Tr) + 1)/2 from t=0 to t=Tr
  Time : Inport
  Add1 : Sum
  Add2 : Sum
  Constant1 : Constant  Value=1/2
  Constant2 : Constant
  Constant3 : Constant  Value=3*pi/2
  Constant4 : Constant  Value=pi
  Divide : Product  Inputs=*/
  Product1 : Product
  Product2 : Product
  Ramp Time : Constant  Value=simu.rampTime
  Sine Wave Function : Sin  TimeSource=Use external signal  SampleTime=0
  R : Outport
  wires:
  Constant1/1 -> Product1/2
  Sine Wave Function/1 -> Add1/2
  Time/1 -> Product2/1
  Product2/1 -> Add2/1
  Add2/1 -> Sine Wave Function/1
  Constant4/1 -> Divide/1
  Add1/1 -> Product1/1
  Divide/1 -> Product2/2  "frequency"
  Ramp Time/1 -> Divide/2  "t_ramp"
  Constant3/1 -> Add2/2  "phase"
  Constant2/1 -> Add1/1
  Product1/1 -> R/1

== system WECSim_Lib_Body_Elements/Flex Body/Wave Radiation Forces Calculation/Wave Radiation Forces Calculation/SS CI and Constant-Damping-CoeVariant Subsystem ==
  note: 1) Add Subsystem or Model blocks as valid variant choices.
      | 2) You cannot connect blocks at this level. At simulation, connectivity is automatically
      | determined, based on the active variant and port name matching.
  note: If the wave type is 'noWave' or 'regular' use constant coefficients.
      | If another wave type and simu.Calc ~= 1, use convolution integral calculation
      | If another wave type and simu.Calc == 1, use the state space calculation
      | If another wave type and simu.FIR == 1, use the FIR filter calculation
  velocity : Inport
  Constant Coefficients : Subsystem  VariantControl=sv_constantCoeff
  Convolution Integral Calculation : Subsystem  VariantControl=sv_convolution
  FIR Filter Calculation : Subsystem  VariantControl=sv_FIR
  "State-Space Calculation " : Subsystem  VariantControl=sv_stateSpace
  Out1 : Outport
